simulink model "filtre_kalman"  (R2019b)
settings: Solver=VariableStepAuto  StartTime=0.0  StopTime=10.0  RelTol=1e-3
values from neighbouring files (symbols this model uses):
  G = 0.002    [Essai_boucle_ouverte.mat]    (also in PAR_PAL1_IDENT.m; mncarres_incomplet.m; mthgraph.m)
undefined symbols (not defined in the file or in its folder): F, H, Kf
settings Model: Creator=ELEPALAN  LastModifiedBy=ELE4202-200
settings DebuggingCC: UnconnectedInputMsg=none  UnconnectedOutputMsg=none  UnconnectedLineMsg=none  SFMachineParentedDataDiag=error

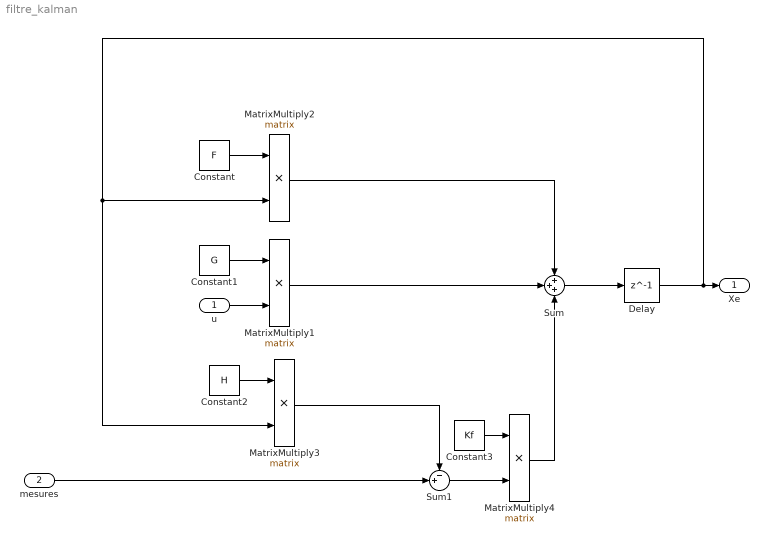
== system filtre_kalman ==
  u : Inport
  mesures : Inport  Port=2
  Constant : Constant  Value=F  SampleTime=-1
  Constant1 : Constant  Value=G  SampleTime=-1
  Constant2 : Constant  Value=H  SampleTime=-1
  Constant3 : Constant  Value=Kf  SampleTime=-1
  Delay : Delay  DelayLength=1
  MatrixMultiply{1..4} (4 alike) : Product  Multiplication=Matrix(*)  SaturateOnIntegerOverflow=on  RndMeth=Zero  InputSameDT=on  OutDataTypeStr=Inherit: Same as first input
  Sum : Sum  Inputs=+++  SaturateOnIntegerOverflow=on  InputSameDT=on  OutDataTypeStr=Inherit: Same as first input
  Sum1 : Sum  Inputs=-+|  SaturateOnIntegerOverflow=on  InputSameDT=on  OutDataTypeStr=Inherit: Same as first input
  Xe : Outport
  wires:
  Constant3/1 -> MatrixMultiply4/1
  MatrixMultiply1/1 -> Sum/2
  MatrixMultiply4/1 -> Sum/3
  mesures/1 -> Sum1/2
  MatrixMultiply3/1 -> Sum1/1
  Sum1/1 -> MatrixMultiply4/2
  Sum/1 -> Delay/1
  Constant/1 -> MatrixMultiply2/1
  Delay/1 -> MatrixMultiply3/2, MatrixMultiply2/2, Xe/1
  Constant2/1 -> MatrixMultiply3/1
  u/1 -> MatrixMultiply1/2
  Constant1/1 -> MatrixMultiply1/1
  MatrixMultiply2/1 -> Sum/1
